simulink model "MMC_21_Level_Rectifier"  (R2023b)
settings: Solver=FixedStepAuto  StartTime=0.0  StopTime=0.5  RelTol=1e-3
libraries: spsSeriesRLCBranchLib x71, spsVoltageMeasurementLib x69, spsUniversalBridgeLib x60, spsCurrentMeasurementLib x8, slpidlib x7, spsRMSLib x3, spsACVoltageSourceLib x3, spsMeanLib x2, simulink x1, spsTHDLib x1, spspowerguiLib x1
(part 2 of 4)

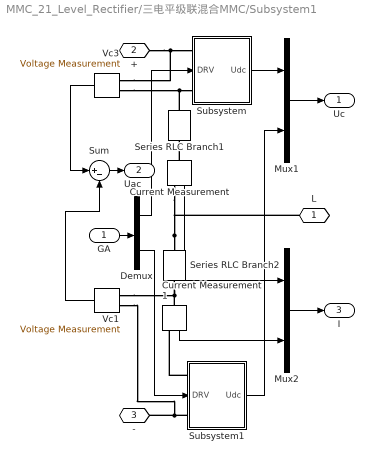
== system MMC_21_Level_Rectifier/三电平级联混合MMC/Subsystem1 ==
  GA : Inport
  Current Measurement : spsCurrentMeasurementLib/Current Measurement  PhasorSimulation=off  OutputType=Complex  PSBequivalent=0
  Current Measurement1 : spsCurrentMeasurementLib/Current Measurement  PhasorSimulation=off  OutputType=Complex  PSBequivalent=0
  Demux : Demux  Outputs=2
  Mux1 : Mux  Inputs=2
  Mux2 : Mux  Inputs=2
  Series RLC Branch1 : spsSeriesRLCBranchLib/Series RLC Branch  LConnTagsString=__new0  RConnTagsString=__new0  BranchType=L  Resistance=30  Inductance=1e-2  SetiL0=off  InitialCurrent=0  Capacitance=1e-6  Setx0=off  InitialVoltage=0  Measurements=None
  Series RLC Branch2 : spsSeriesRLCBranchLib/Series RLC Branch  LConnTagsString=__new0  RConnTagsString=__new0  BranchType=L  Resistance=30  Inductance=1e-2  SetiL0=off  InitialCurrent=0  Capacitance=1e-6  Setx0=off  InitialVoltage=0  Measurements=None
  Subsystem : Subsystem
      settings: PortSchema="{\"entries\":[{\"content\":{\"sides\":[{\"content\":{\"connectorIds\":[\"LConn1\",\"In1\",\"LConn2\"]},\"type\":\"ConnectorPlacement.EquallySpacedRectSide\",\"uuid\":\"6ff65170-2c54-424c-bb24-a96dc10d43f1\"},{\"content\":{\"connectorIds\":[\"Out1\"],\"side\":\"RIGHT\"},\"type\":\"ConnectorPlacement.EquallySpacedRectSide\",\"uuid\":\"90bd0adf-4df3-4011-8d6e-6638ef6b0231\"},{\"content\":{\"side\":\"TOP\"},\"type\":\"ConnectorPlacement.EquallySpacedRectSide\",\"uuid\":\"3c2ececc-9eb8-4d9a-8cd6-b7f9ee8fbc54\"}]},\"type\":\"ConnectorPlacement.EquallySpacedConnector\",\"uuid\":\"28e6b26b-947d-4977-abd9-a0ec0787b735\"}],\"packageUris\":[\"http://schema.mathworks.com/mf0/Connector/R2020b\"],\"version\":\"1.0\"}"
  Subsystem1 : Subsystem
      settings: PortSchema="{\"entries\":[{\"content\":{\"sides\":[{\"content\":{\"connectorIds\":[\"LConn1\",\"In1\",\"LConn2\"]},\"type\":\"ConnectorPlacement.EquallySpacedRectSide\",\"uuid\":\"6ff65170-2c54-424c-bb24-a96dc10d43f1\"},{\"content\":{\"connectorIds\":[\"Out1\"],\"side\":\"RIGHT\"},\"type\":\"ConnectorPlacement.EquallySpacedRectSide\",\"uuid\":\"90bd0adf-4df3-4011-8d6e-6638ef6b0231\"},{\"content\":{\"side\":\"TOP\"},\"type\":\"ConnectorPlacement.EquallySpacedRectSide\",\"uuid\":\"3c2ececc-9eb8-4d9a-8cd6-b7f9ee8fbc54\"}]},\"type\":\"ConnectorPlacement.EquallySpacedConnector\",\"uuid\":\"28e6b26b-947d-4977-abd9-a0ec0787b735\"}],\"packageUris\":[\"http://schema.mathworks.com/mf0/Connector/R2020b\"],\"version\":\"1.0\"}"
  Sum : Sum  Inputs=|+-
  Vc1 : spsVoltageMeasurementLib/Voltage Measurement  PhasorSimulation=off  OutputType=Complex  PSBequivalent=0
  Vc3 : spsVoltageMeasurementLib/Voltage Measurement  PhasorSimulation=off  OutputType=Complex  PSBequivalent=0
  L : PMIOPort  Side=Left
  + : PMIOPort  Port=2  Side=Left
  - : PMIOPort  Port=3  Side=Right
  Uc : Outport
  Uac : Outport  Port=2
  I : Outport  Port=3
  wires:
  Sum/1 -> Uac/1
  Vc1/1 -> Sum/2
  Vc3/1 -> Sum/1
  Mux2/1 -> I/1
  Current Measurement1/1 -> Mux2/2
  GA/1 -> Demux/1
  Demux/1 -> Subsystem/1(DRV)
  Current Measurement/1 -> Mux2/1
  Subsystem/1(Udc) -> Mux1/1
  Mux1/1 -> Uc/1
  Subsystem1/1(Udc) -> Mux1/2
  Demux/2 -> Subsystem1/1(DRV)
  connections:
  Vc1/LConn1 -- Series RLC Branch2/RConn1 -- Current Measurement1/LConn1
  Vc3/LConn1 -- +/RConn1 -- Subsystem/LConn1
  Vc1/LConn2 -- Subsystem1/LConn2 -- -/RConn1
  Current Measurement/LConn1 -- Series RLC Branch1/RConn1
  Subsystem1/LConn1 -- Current Measurement1/RConn1
  Subsystem/LConn2 -- Vc3/LConn2 -- Series RLC Branch1/LConn1
  Series RLC Branch2/LConn1 -- L/RConn1 -- Current Measurement/RConn1

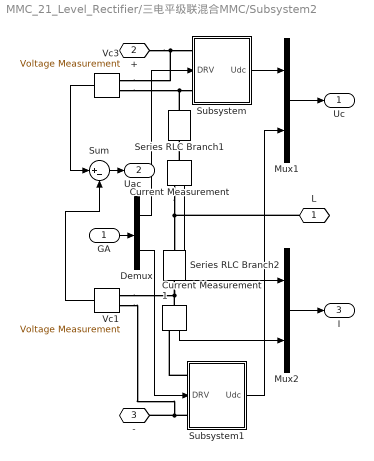
== system MMC_21_Level_Rectifier/三电平级联混合MMC/Subsystem2 ==
  GA : Inport
  Current Measurement : spsCurrentMeasurementLib/Current Measurement  PhasorSimulation=off  OutputType=Complex  PSBequivalent=0
  Current Measurement1 : spsCurrentMeasurementLib/Current Measurement  PhasorSimulation=off  OutputType=Complex  PSBequivalent=0
  Demux : Demux  Outputs=2
  Mux1 : Mux  Inputs=2
  Mux2 : Mux  Inputs=2
  Series RLC Branch1 : spsSeriesRLCBranchLib/Series RLC Branch  LConnTagsString=__new0  RConnTagsString=__new0  BranchType=L  Resistance=30  Inductance=1e-2  SetiL0=off  InitialCurrent=0  Capacitance=1e-6  Setx0=off  InitialVoltage=0  Measurements=None
  Series RLC Branch2 : spsSeriesRLCBranchLib/Series RLC Branch  LConnTagsString=__new0  RConnTagsString=__new0  BranchType=L  Resistance=30  Inductance=1e-2  SetiL0=off  InitialCurrent=0  Capacitance=1e-6  Setx0=off  InitialVoltage=0  Measurements=None
  Subsystem : Subsystem
      settings: PortSchema="{\"entries\":[{\"content\":{\"sides\":[{\"content\":{\"connectorIds\":[\"LConn1\",\"In1\",\"LConn2\"]},\"type\":\"ConnectorPlacement.EquallySpacedRectSide\",\"uuid\":\"6ff65170-2c54-424c-bb24-a96dc10d43f1\"},{\"content\":{\"connectorIds\":[\"Out1\"],\"side\":\"RIGHT\"},\"type\":\"ConnectorPlacement.EquallySpacedRectSide\",\"uuid\":\"90bd0adf-4df3-4011-8d6e-6638ef6b0231\"},{\"content\":{\"side\":\"TOP\"},\"type\":\"ConnectorPlacement.EquallySpacedRectSide\",\"uuid\":\"3c2ececc-9eb8-4d9a-8cd6-b7f9ee8fbc54\"}]},\"type\":\"ConnectorPlacement.EquallySpacedConnector\",\"uuid\":\"28e6b26b-947d-4977-abd9-a0ec0787b735\"}],\"packageUris\":[\"http://schema.mathworks.com/mf0/Connector/R2020b\"],\"version\":\"1.0\"}"
  Subsystem1 : Subsystem
      settings: PortSchema="{\"entries\":[{\"content\":{\"sides\":[{\"content\":{\"connectorIds\":[\"LConn1\",\"In1\",\"LConn2\"]},\"type\":\"ConnectorPlacement.EquallySpacedRectSide\",\"uuid\":\"6ff65170-2c54-424c-bb24-a96dc10d43f1\"},{\"content\":{\"connectorIds\":[\"Out1\"],\"side\":\"RIGHT\"},\"type\":\"ConnectorPlacement.EquallySpacedRectSide\",\"uuid\":\"90bd0adf-4df3-4011-8d6e-6638ef6b0231\"},{\"content\":{\"side\":\"TOP\"},\"type\":\"ConnectorPlacement.EquallySpacedRectSide\",\"uuid\":\"3c2ececc-9eb8-4d9a-8cd6-b7f9ee8fbc54\"}]},\"type\":\"ConnectorPlacement.EquallySpacedConnector\",\"uuid\":\"28e6b26b-947d-4977-abd9-a0ec0787b735\"}],\"packageUris\":[\"http://schema.mathworks.com/mf0/Connector/R2020b\"],\"version\":\"1.0\"}"
  Sum : Sum  Inputs=|+-
  Vc1 : spsVoltageMeasurementLib/Voltage Measurement  PhasorSimulation=off  OutputType=Complex  PSBequivalent=0
  Vc3 : spsVoltageMeasurementLib/Voltage Measurement  PhasorSimulation=off  OutputType=Complex  PSBequivalent=0
  L : PMIOPort  Side=Left
  + : PMIOPort  Port=2  Side=Left
  - : PMIOPort  Port=3  Side=Right
  Uc : Outport
  Uac : Outport  Port=2
  I : Outport  Port=3
  wires:
  Demux/2 -> Subsystem1/1(DRV)
  Subsystem1/1(Udc) -> Mux1/2
  Mux1/1 -> Uc/1
  Subsystem/1(Udc) -> Mux1/1
  Current Measurement/1 -> Mux2/1
  Demux/1 -> Subsystem/1(DRV)
  GA/1 -> Demux/1
  Current Measurement1/1 -> Mux2/2
  Mux2/1 -> I/1
  Vc3/1 -> Sum/1
  Vc1/1 -> Sum/2
  Sum/1 -> Uac/1
  connections:
  Current Measurement/RConn1 -- Series RLC Branch2/LConn1 -- L/RConn1
  Series RLC Branch1/LConn1 -- Vc3/LConn2 -- Subsystem/LConn2
  Subsystem1/LConn1 -- Current Measurement1/RConn1
  Current Measurement/LConn1 -- Series RLC Branch1/RConn1
  Subsystem1/LConn2 -- Vc1/LConn2 -- -/RConn1
  +/RConn1 -- Vc3/LConn1 -- Subsystem/LConn1
  Current Measurement1/LConn1 -- Vc1/LConn1 -- Series RLC Branch2/RConn1

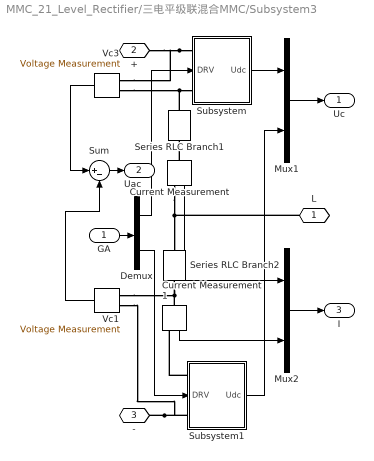
== system MMC_21_Level_Rectifier/三电平级联混合MMC/Subsystem3 ==
  GA : Inport
  Current Measurement : spsCurrentMeasurementLib/Current Measurement  PhasorSimulation=off  OutputType=Complex  PSBequivalent=0
  Current Measurement1 : spsCurrentMeasurementLib/Current Measurement  PhasorSimulation=off  OutputType=Complex  PSBequivalent=0
  Demux : Demux  Outputs=2
  Mux1 : Mux  Inputs=2
  Mux2 : Mux  Inputs=2
  Series RLC Branch1 : spsSeriesRLCBranchLib/Series RLC Branch  LConnTagsString=__new0  RConnTagsString=__new0  BranchType=L  Resistance=30  Inductance=1e-2  SetiL0=off  InitialCurrent=0  Capacitance=1e-6  Setx0=off  InitialVoltage=0  Measurements=None
  Series RLC Branch2 : spsSeriesRLCBranchLib/Series RLC Branch  LConnTagsString=__new0  RConnTagsString=__new0  BranchType=L  Resistance=30  Inductance=1e-2  SetiL0=off  InitialCurrent=0  Capacitance=1e-6  Setx0=off  InitialVoltage=0  Measurements=None
  Subsystem : Subsystem
      settings: PortSchema="{\"entries\":[{\"content\":{\"sides\":[{\"content\":{\"connectorIds\":[\"LConn1\",\"In1\",\"LConn2\"]},\"type\":\"ConnectorPlacement.EquallySpacedRectSide\",\"uuid\":\"6ff65170-2c54-424c-bb24-a96dc10d43f1\"},{\"content\":{\"connectorIds\":[\"Out1\"],\"side\":\"RIGHT\"},\"type\":\"ConnectorPlacement.EquallySpacedRectSide\",\"uuid\":\"90bd0adf-4df3-4011-8d6e-6638ef6b0231\"},{\"content\":{\"side\":\"TOP\"},\"type\":\"ConnectorPlacement.EquallySpacedRectSide\",\"uuid\":\"3c2ececc-9eb8-4d9a-8cd6-b7f9ee8fbc54\"}]},\"type\":\"ConnectorPlacement.EquallySpacedConnector\",\"uuid\":\"28e6b26b-947d-4977-abd9-a0ec0787b735\"}],\"packageUris\":[\"http://schema.mathworks.com/mf0/Connector/R2020b\"],\"version\":\"1.0\"}"
  Subsystem1 : Subsystem
      settings: PortSchema="{\"entries\":[{\"content\":{\"sides\":[{\"content\":{\"connectorIds\":[\"LConn1\",\"In1\",\"LConn2\"]},\"type\":\"ConnectorPlacement.EquallySpacedRectSide\",\"uuid\":\"6ff65170-2c54-424c-bb24-a96dc10d43f1\"},{\"content\":{\"connectorIds\":[\"Out1\"],\"side\":\"RIGHT\"},\"type\":\"ConnectorPlacement.EquallySpacedRectSide\",\"uuid\":\"90bd0adf-4df3-4011-8d6e-6638ef6b0231\"},{\"content\":{\"side\":\"TOP\"},\"type\":\"ConnectorPlacement.EquallySpacedRectSide\",\"uuid\":\"3c2ececc-9eb8-4d9a-8cd6-b7f9ee8fbc54\"}]},\"type\":\"ConnectorPlacement.EquallySpacedConnector\",\"uuid\":\"28e6b26b-947d-4977-abd9-a0ec0787b735\"}],\"packageUris\":[\"http://schema.mathworks.com/mf0/Connector/R2020b\"],\"version\":\"1.0\"}"
  Sum : Sum  Inputs=|+-
  Vc1 : spsVoltageMeasurementLib/Voltage Measurement  PhasorSimulation=off  OutputType=Complex  PSBequivalent=0
  Vc3 : spsVoltageMeasurementLib/Voltage Measurement  PhasorSimulation=off  OutputType=Complex  PSBequivalent=0
  L : PMIOPort  Side=Left
  + : PMIOPort  Port=2  Side=Left
  - : PMIOPort  Port=3  Side=Right
  Uc : Outport
  Uac : Outport  Port=2
  I : Outport  Port=3
  wires:
  Demux/2 -> Subsystem1/1(DRV)
  Subsystem1/1(Udc) -> Mux1/2
  Mux1/1 -> Uc/1
  Subsystem/1(Udc) -> Mux1/1
  Current Measurement/1 -> Mux2/1
  Demux/1 -> Subsystem/1(DRV)
  GA/1 -> Demux/1
  Current Measurement1/1 -> Mux2/2
  Mux2/1 -> I/1
  Vc3/1 -> Sum/1
  Vc1/1 -> Sum/2
  Sum/1 -> Uac/1
  connections:
  Current Measurement/RConn1 -- L/RConn1 -- Series RLC Branch2/LConn1
  Series RLC Branch1/LConn1 -- Vc3/LConn2 -- Subsystem/LConn2
  Subsystem1/LConn1 -- Current Measurement1/RConn1
  Current Measurement/LConn1 -- Series RLC Branch1/RConn1
  -/RConn1 -- Subsystem1/LConn2 -- Vc1/LConn2
  Subsystem/LConn1 -- +/RConn1 -- Vc3/LConn1
  Current Measurement1/LConn1 -- Series RLC Branch2/RConn1 -- Vc1/LConn1

== system MMC_21_Level_Rectifier/准PR电压电流环路/2//3 Transform ==
  ac : Inport
  Demux : Demux  Outputs=2
  Mux : Mux  Inputs=3
  Sum1 : Sum  Inputs=-|-
  abc : Outport
  wires:
  Sum1/1 -> Mux/2
  Mux/1 -> abc/1
  Demux/1 -> Sum1/1, Mux/1
  ac/1 -> Demux/1
  Demux/2 -> Sum1/2, Mux/3

== system MMC_21_Level_Rectifier/准PR电压电流环路/Digital PR A-C ==
  err : Inport
  Constant : Constant  Value=Kp
  Constant1 : Constant  Value=Kr
  Constant2 : Constant  Value=Wc
  Constant3 : Constant  Value=Ts
  Demux : Demux  Outputs=2
  Discrete PR : MATLAB Function  TreatAsAtomicUnit=on
  Mux : Mux  Inputs=2
  Saturation : Saturate  UpperLimit=Upper  LowerLimit=Lower
  out : Outport
  wires:
  Constant1/1 -> Discrete PR/4(Kr)
  Constant3/1 -> Discrete PR/6(Ts)
  Constant/1 -> Discrete PR/3(Kp)
  Constant2/1 -> Discrete PR/5(Wc)
  Demux/1 -> Discrete PR/1(err_A)
  err/1 -> Demux/1
  Demux/2 -> Discrete PR/2(err_C)
  Discrete PR/1(out_A) -> Mux/1
  Discrete PR/2(out_C) -> Mux/2
  Mux/1 -> Saturation/1
  Saturation/1 -> out/1

== system MMC_21_Level_Rectifier/三电平级联混合MMC/Subsystem1/Subsystem ==
  DRV : Inport
  Demux1 : Demux  Outputs=5
  Mux1 : Mux  Inputs=5
  混合三电平子模块1 : Subsystem
      settings: PortSchema="{\"entries\":[{\"content\":{\"sides\":[{\"content\":{\"connectorIds\":[\"LConn1\",\"In1\",\"LConn2\"]},\"type\":\"ConnectorPlacement.EquallySpacedRectSide\",\"uuid\":\"9e595762-cb5d-4bdb-b148-c61b2a1e03b2\"},{\"content\":{\"connectorIds\":[\"Out1\"],\"side\":\"RIGHT\"},\"type\":\"ConnectorPlacement.EquallySpacedRectSide\",\"uuid\":\"493db82a-06a2-4a87-b234-4e7c0dd8f89b\"},{\"content\":{\"side\":\"TOP\"},\"type\":\"ConnectorPlacement.EquallySpacedRectSide\",\"uuid\":\"00eff750-16ab-4a5d-887e-7c480e5e0d14\"}]},\"type\":\"ConnectorPlacement.EquallySpacedConnector\",\"uuid\":\"9358f970-c1dc-48f9-b6f8-bcc3c6345ab1\"}],\"packageUris\":[\"http://schema.mathworks.com/mf0/Connector/R2020b\"],\"version\":\"1.0\"}"
  混合三电平子模块2 : Subsystem
      settings: PortSchema="{\"entries\":[{\"content\":{\"sides\":[{\"content\":{\"connectorIds\":[\"LConn1\",\"In1\",\"LConn2\"]},\"type\":\"ConnectorPlacement.EquallySpacedRectSide\",\"uuid\":\"9e595762-cb5d-4bdb-b148-c61b2a1e03b2\"},{\"content\":{\"connectorIds\":[\"Out1\"],\"side\":\"RIGHT\"},\"type\":\"ConnectorPlacement.EquallySpacedRectSide\",\"uuid\":\"493db82a-06a2-4a87-b234-4e7c0dd8f89b\"},{\"content\":{\"side\":\"TOP\"},\"type\":\"ConnectorPlacement.EquallySpacedRectSide\",\"uuid\":\"00eff750-16ab-4a5d-887e-7c480e5e0d14\"}]},\"type\":\"ConnectorPlacement.EquallySpacedConnector\",\"uuid\":\"9358f970-c1dc-48f9-b6f8-bcc3c6345ab1\"}],\"packageUris\":[\"http://schema.mathworks.com/mf0/Connector/R2020b\"],\"version\":\"1.0\"}"
  混合三电平子模块3 : Subsystem
      settings: PortSchema="{\"entries\":[{\"content\":{\"sides\":[{\"content\":{\"connectorIds\":[\"LConn1\",\"In1\",\"LConn2\"]},\"type\":\"ConnectorPlacement.EquallySpacedRectSide\",\"uuid\":\"9e595762-cb5d-4bdb-b148-c61b2a1e03b2\"},{\"content\":{\"connectorIds\":[\"Out1\"],\"side\":\"RIGHT\"},\"type\":\"ConnectorPlacement.EquallySpacedRectSide\",\"uuid\":\"493db82a-06a2-4a87-b234-4e7c0dd8f89b\"},{\"content\":{\"side\":\"TOP\"},\"type\":\"ConnectorPlacement.EquallySpacedRectSide\",\"uuid\":\"00eff750-16ab-4a5d-887e-7c480e5e0d14\"}]},\"type\":\"ConnectorPlacement.EquallySpacedConnector\",\"uuid\":\"9358f970-c1dc-48f9-b6f8-bcc3c6345ab1\"}],\"packageUris\":[\"http://schema.mathworks.com/mf0/Connector/R2020b\"],\"version\":\"1.0\"}"
  混合三电平子模块4 : Subsystem
      settings: PortSchema="{\"entries\":[{\"content\":{\"sides\":[{\"content\":{\"connectorIds\":[\"LConn1\",\"In1\",\"LConn2\"]},\"type\":\"ConnectorPlacement.EquallySpacedRectSide\",\"uuid\":\"9e595762-cb5d-4bdb-b148-c61b2a1e03b2\"},{\"content\":{\"connectorIds\":[\"Out1\"],\"side\":\"RIGHT\"},\"type\":\"ConnectorPlacement.EquallySpacedRectSide\",\"uuid\":\"493db82a-06a2-4a87-b234-4e7c0dd8f89b\"},{\"content\":{\"side\":\"TOP\"},\"type\":\"ConnectorPlacement.EquallySpacedRectSide\",\"uuid\":\"00eff750-16ab-4a5d-887e-7c480e5e0d14\"}]},\"type\":\"ConnectorPlacement.EquallySpacedConnector\",\"uuid\":\"9358f970-c1dc-48f9-b6f8-bcc3c6345ab1\"}],\"packageUris\":[\"http://schema.mathworks.com/mf0/Connector/R2020b\"],\"version\":\"1.0\"}"
  混合三电平子模块5 : Subsystem
      settings: PortSchema="{\"entries\":[{\"content\":{\"sides\":[{\"content\":{\"connectorIds\":[\"LConn1\",\"In1\",\"LConn2\"]},\"type\":\"ConnectorPlacement.EquallySpacedRectSide\",\"uuid\":\"9e595762-cb5d-4bdb-b148-c61b2a1e03b2\"},{\"content\":{\"connectorIds\":[\"Out1\"],\"side\":\"RIGHT\"},\"type\":\"ConnectorPlacement.EquallySpacedRectSide\",\"uuid\":\"493db82a-06a2-4a87-b234-4e7c0dd8f89b\"},{\"content\":{\"side\":\"TOP\"},\"type\":\"ConnectorPlacement.EquallySpacedRectSide\",\"uuid\":\"00eff750-16ab-4a5d-887e-7c480e5e0d14\"}]},\"type\":\"ConnectorPlacement.EquallySpacedConnector\",\"uuid\":\"9358f970-c1dc-48f9-b6f8-bcc3c6345ab1\"}],\"packageUris\":[\"http://schema.mathworks.com/mf0/Connector/R2020b\"],\"version\":\"1.0\"}"
  + : PMIOPort  Side=Left
  - : PMIOPort  Port=2  Side=Left
  Udc : Outport
  wires:
  混合三电平子模块1/1(Udc) -> Mux1/1
  Mux1/1 -> Udc/1
  混合三电平子模块5/1(Udc) -> Mux1/5
  混合三电平子模块4/1(Udc) -> Mux1/4
  混合三电平子模块2/1(Udc) -> Mux1/2
  混合三电平子模块3/1(Udc) -> Mux1/3
  Demux1/5 -> 混合三电平子模块5/1(DRV)
  Demux1/4 -> 混合三电平子模块4/1(DRV)
  Demux1/2 -> 混合三电平子模块2/1(DRV)
  Demux1/3 -> 混合三电平子模块3/1(DRV)
  Demux1/1 -> 混合三电平子模块1/1(DRV)
  DRV/1 -> Demux1/1
  connections:
  混合三电平子模块5/LConn1 -- 混合三电平子模块4/LConn2
  混合三电平子模块4/LConn1 -- 混合三电平子模块3/LConn2
  混合三电平子模块3/LConn1 -- 混合三电平子模块2/LConn2
  混合三电平子模块2/LConn1 -- 混合三电平子模块1/LConn2
  +/RConn1 -- 混合三电平子模块1/LConn1
  混合三电平子模块5/LConn2 -- -/RConn1

== system MMC_21_Level_Rectifier/三电平级联混合MMC/Subsystem1/Subsystem1 ==
  DRV : Inport
  Demux1 : Demux  Outputs=5
  Mux1 : Mux  Inputs=5
  混合三电平子模块1 : Subsystem
      settings: PortSchema="{\"entries\":[{\"content\":{\"sides\":[{\"content\":{\"connectorIds\":[\"LConn1\",\"In1\",\"LConn2\"]},\"type\":\"ConnectorPlacement.EquallySpacedRectSide\",\"uuid\":\"9e595762-cb5d-4bdb-b148-c61b2a1e03b2\"},{\"content\":{\"connectorIds\":[\"Out1\"],\"side\":\"RIGHT\"},\"type\":\"ConnectorPlacement.EquallySpacedRectSide\",\"uuid\":\"493db82a-06a2-4a87-b234-4e7c0dd8f89b\"},{\"content\":{\"side\":\"TOP\"},\"type\":\"ConnectorPlacement.EquallySpacedRectSide\",\"uuid\":\"00eff750-16ab-4a5d-887e-7c480e5e0d14\"}]},\"type\":\"ConnectorPlacement.EquallySpacedConnector\",\"uuid\":\"9358f970-c1dc-48f9-b6f8-bcc3c6345ab1\"}],\"packageUris\":[\"http://schema.mathworks.com/mf0/Connector/R2020b\"],\"version\":\"1.0\"}"
  混合三电平子模块2 : Subsystem
      settings: PortSchema="{\"entries\":[{\"content\":{\"sides\":[{\"content\":{\"connectorIds\":[\"LConn1\",\"In1\",\"LConn2\"]},\"type\":\"ConnectorPlacement.EquallySpacedRectSide\",\"uuid\":\"9e595762-cb5d-4bdb-b148-c61b2a1e03b2\"},{\"content\":{\"connectorIds\":[\"Out1\"],\"side\":\"RIGHT\"},\"type\":\"ConnectorPlacement.EquallySpacedRectSide\",\"uuid\":\"493db82a-06a2-4a87-b234-4e7c0dd8f89b\"},{\"content\":{\"side\":\"TOP\"},\"type\":\"ConnectorPlacement.EquallySpacedRectSide\",\"uuid\":\"00eff750-16ab-4a5d-887e-7c480e5e0d14\"}]},\"type\":\"ConnectorPlacement.EquallySpacedConnector\",\"uuid\":\"9358f970-c1dc-48f9-b6f8-bcc3c6345ab1\"}],\"packageUris\":[\"http://schema.mathworks.com/mf0/Connector/R2020b\"],\"version\":\"1.0\"}"
  混合三电平子模块3 : Subsystem
      settings: PortSchema="{\"entries\":[{\"content\":{\"sides\":[{\"content\":{\"connectorIds\":[\"LConn1\",\"In1\",\"LConn2\"]},\"type\":\"ConnectorPlacement.EquallySpacedRectSide\",\"uuid\":\"9e595762-cb5d-4bdb-b148-c61b2a1e03b2\"},{\"content\":{\"connectorIds\":[\"Out1\"],\"side\":\"RIGHT\"},\"type\":\"ConnectorPlacement.EquallySpacedRectSide\",\"uuid\":\"493db82a-06a2-4a87-b234-4e7c0dd8f89b\"},{\"content\":{\"side\":\"TOP\"},\"type\":\"ConnectorPlacement.EquallySpacedRectSide\",\"uuid\":\"00eff750-16ab-4a5d-887e-7c480e5e0d14\"}]},\"type\":\"ConnectorPlacement.EquallySpacedConnector\",\"uuid\":\"9358f970-c1dc-48f9-b6f8-bcc3c6345ab1\"}],\"packageUris\":[\"http://schema.mathworks.com/mf0/Connector/R2020b\"],\"version\":\"1.0\"}"
  混合三电平子模块4 : Subsystem
      settings: PortSchema="{\"entries\":[{\"content\":{\"sides\":[{\"content\":{\"connectorIds\":[\"LConn1\",\"In1\",\"LConn2\"]},\"type\":\"ConnectorPlacement.EquallySpacedRectSide\",\"uuid\":\"9e595762-cb5d-4bdb-b148-c61b2a1e03b2\"},{\"content\":{\"connectorIds\":[\"Out1\"],\"side\":\"RIGHT\"},\"type\":\"ConnectorPlacement.EquallySpacedRectSide\",\"uuid\":\"493db82a-06a2-4a87-b234-4e7c0dd8f89b\"},{\"content\":{\"side\":\"TOP\"},\"type\":\"ConnectorPlacement.EquallySpacedRectSide\",\"uuid\":\"00eff750-16ab-4a5d-887e-7c480e5e0d14\"}]},\"type\":\"ConnectorPlacement.EquallySpacedConnector\",\"uuid\":\"9358f970-c1dc-48f9-b6f8-bcc3c6345ab1\"}],\"packageUris\":[\"http://schema.mathworks.com/mf0/Connector/R2020b\"],\"version\":\"1.0\"}"
  混合三电平子模块5 : Subsystem
      settings: PortSchema="{\"entries\":[{\"content\":{\"sides\":[{\"content\":{\"connectorIds\":[\"LConn1\",\"In1\",\"LConn2\"]},\"type\":\"ConnectorPlacement.EquallySpacedRectSide\",\"uuid\":\"9e595762-cb5d-4bdb-b148-c61b2a1e03b2\"},{\"content\":{\"connectorIds\":[\"Out1\"],\"side\":\"RIGHT\"},\"type\":\"ConnectorPlacement.EquallySpacedRectSide\",\"uuid\":\"493db82a-06a2-4a87-b234-4e7c0dd8f89b\"},{\"content\":{\"side\":\"TOP\"},\"type\":\"ConnectorPlacement.EquallySpacedRectSide\",\"uuid\":\"00eff750-16ab-4a5d-887e-7c480e5e0d14\"}]},\"type\":\"ConnectorPlacement.EquallySpacedConnector\",\"uuid\":\"9358f970-c1dc-48f9-b6f8-bcc3c6345ab1\"}],\"packageUris\":[\"http://schema.mathworks.com/mf0/Connector/R2020b\"],\"version\":\"1.0\"}"
  + : PMIOPort  Side=Left
  - : PMIOPort  Port=2  Side=Left
  Udc : Outport
  wires:
  DRV/1 -> Demux1/1
  Demux1/1 -> 混合三电平子模块1/1(DRV)
  Demux1/3 -> 混合三电平子模块3/1(DRV)
  Demux1/2 -> 混合三电平子模块2/1(DRV)
  Demux1/4 -> 混合三电平子模块4/1(DRV)
  Demux1/5 -> 混合三电平子模块5/1(DRV)
  混合三电平子模块3/1(Udc) -> Mux1/3
  混合三电平子模块2/1(Udc) -> Mux1/2
  混合三电平子模块4/1(Udc) -> Mux1/4
  混合三电平子模块5/1(Udc) -> Mux1/5
  Mux1/1 -> Udc/1
  混合三电平子模块1/1(Udc) -> Mux1/1
  connections:
  混合三电平子模块5/LConn2 -- -/RConn1
  +/RConn1 -- 混合三电平子模块1/LConn1
  混合三电平子模块2/LConn1 -- 混合三电平子模块1/LConn2
  混合三电平子模块3/LConn1 -- 混合三电平子模块2/LConn2
  混合三电平子模块4/LConn1 -- 混合三电平子模块3/LConn2
  混合三电平子模块5/LConn1 -- 混合三电平子模块4/LConn2

== system MMC_21_Level_Rectifier/三电平级联混合MMC/Subsystem2/Subsystem ==
  DRV : Inport
  Demux1 : Demux  Outputs=5
  Mux1 : Mux  Inputs=5
  混合三电平子模块1 : Subsystem
      settings: PortSchema="{\"entries\":[{\"content\":{\"sides\":[{\"content\":{\"connectorIds\":[\"LConn1\",\"In1\",\"LConn2\"]},\"type\":\"ConnectorPlacement.EquallySpacedRectSide\",\"uuid\":\"9e595762-cb5d-4bdb-b148-c61b2a1e03b2\"},{\"content\":{\"connectorIds\":[\"Out1\"],\"side\":\"RIGHT\"},\"type\":\"ConnectorPlacement.EquallySpacedRectSide\",\"uuid\":\"493db82a-06a2-4a87-b234-4e7c0dd8f89b\"},{\"content\":{\"side\":\"TOP\"},\"type\":\"ConnectorPlacement.EquallySpacedRectSide\",\"uuid\":\"00eff750-16ab-4a5d-887e-7c480e5e0d14\"}]},\"type\":\"ConnectorPlacement.EquallySpacedConnector\",\"uuid\":\"9358f970-c1dc-48f9-b6f8-bcc3c6345ab1\"}],\"packageUris\":[\"http://schema.mathworks.com/mf0/Connector/R2020b\"],\"version\":\"1.0\"}"
  混合三电平子模块2 : Subsystem
      settings: PortSchema="{\"entries\":[{\"content\":{\"sides\":[{\"content\":{\"connectorIds\":[\"LConn1\",\"In1\",\"LConn2\"]},\"type\":\"ConnectorPlacement.EquallySpacedRectSide\",\"uuid\":\"9e595762-cb5d-4bdb-b148-c61b2a1e03b2\"},{\"content\":{\"connectorIds\":[\"Out1\"],\"side\":\"RIGHT\"},\"type\":\"ConnectorPlacement.EquallySpacedRectSide\",\"uuid\":\"493db82a-06a2-4a87-b234-4e7c0dd8f89b\"},{\"content\":{\"side\":\"TOP\"},\"type\":\"ConnectorPlacement.EquallySpacedRectSide\",\"uuid\":\"00eff750-16ab-4a5d-887e-7c480e5e0d14\"}]},\"type\":\"ConnectorPlacement.EquallySpacedConnector\",\"uuid\":\"9358f970-c1dc-48f9-b6f8-bcc3c6345ab1\"}],\"packageUris\":[\"http://schema.mathworks.com/mf0/Connector/R2020b\"],\"version\":\"1.0\"}"
  混合三电平子模块3 : Subsystem
      settings: PortSchema="{\"entries\":[{\"content\":{\"sides\":[{\"content\":{\"connectorIds\":[\"LConn1\",\"In1\",\"LConn2\"]},\"type\":\"ConnectorPlacement.EquallySpacedRectSide\",\"uuid\":\"9e595762-cb5d-4bdb-b148-c61b2a1e03b2\"},{\"content\":{\"connectorIds\":[\"Out1\"],\"side\":\"RIGHT\"},\"type\":\"ConnectorPlacement.EquallySpacedRectSide\",\"uuid\":\"493db82a-06a2-4a87-b234-4e7c0dd8f89b\"},{\"content\":{\"side\":\"TOP\"},\"type\":\"ConnectorPlacement.EquallySpacedRectSide\",\"uuid\":\"00eff750-16ab-4a5d-887e-7c480e5e0d14\"}]},\"type\":\"ConnectorPlacement.EquallySpacedConnector\",\"uuid\":\"9358f970-c1dc-48f9-b6f8-bcc3c6345ab1\"}],\"packageUris\":[\"http://schema.mathworks.com/mf0/Connector/R2020b\"],\"version\":\"1.0\"}"
  混合三电平子模块4 : Subsystem
      settings: PortSchema="{\"entries\":[{\"content\":{\"sides\":[{\"content\":{\"connectorIds\":[\"LConn1\",\"In1\",\"LConn2\"]},\"type\":\"ConnectorPlacement.EquallySpacedRectSide\",\"uuid\":\"9e595762-cb5d-4bdb-b148-c61b2a1e03b2\"},{\"content\":{\"connectorIds\":[\"Out1\"],\"side\":\"RIGHT\"},\"type\":\"ConnectorPlacement.EquallySpacedRectSide\",\"uuid\":\"493db82a-06a2-4a87-b234-4e7c0dd8f89b\"},{\"content\":{\"side\":\"TOP\"},\"type\":\"ConnectorPlacement.EquallySpacedRectSide\",\"uuid\":\"00eff750-16ab-4a5d-887e-7c480e5e0d14\"}]},\"type\":\"ConnectorPlacement.EquallySpacedConnector\",\"uuid\":\"9358f970-c1dc-48f9-b6f8-bcc3c6345ab1\"}],\"packageUris\":[\"http://schema.mathworks.com/mf0/Connector/R2020b\"],\"version\":\"1.0\"}"
  混合三电平子模块5 : Subsystem
      settings: PortSchema="{\"entries\":[{\"content\":{\"sides\":[{\"content\":{\"connectorIds\":[\"LConn1\",\"In1\",\"LConn2\"]},\"type\":\"ConnectorPlacement.EquallySpacedRectSide\",\"uuid\":\"9e595762-cb5d-4bdb-b148-c61b2a1e03b2\"},{\"content\":{\"connectorIds\":[\"Out1\"],\"side\":\"RIGHT\"},\"type\":\"ConnectorPlacement.EquallySpacedRectSide\",\"uuid\":\"493db82a-06a2-4a87-b234-4e7c0dd8f89b\"},{\"content\":{\"side\":\"TOP\"},\"type\":\"ConnectorPlacement.EquallySpacedRectSide\",\"uuid\":\"00eff750-16ab-4a5d-887e-7c480e5e0d14\"}]},\"type\":\"ConnectorPlacement.EquallySpacedConnector\",\"uuid\":\"9358f970-c1dc-48f9-b6f8-bcc3c6345ab1\"}],\"packageUris\":[\"http://schema.mathworks.com/mf0/Connector/R2020b\"],\"version\":\"1.0\"}"
  + : PMIOPort  Side=Left
  - : PMIOPort  Port=2  Side=Left
  Udc : Outport
  wires:
  DRV/1 -> Demux1/1
  Demux1/1 -> 混合三电平子模块1/1(DRV)
  Demux1/3 -> 混合三电平子模块3/1(DRV)
  Demux1/2 -> 混合三电平子模块2/1(DRV)
  Demux1/4 -> 混合三电平子模块4/1(DRV)
  Demux1/5 -> 混合三电平子模块5/1(DRV)
  混合三电平子模块3/1(Udc) -> Mux1/3
  混合三电平子模块2/1(Udc) -> Mux1/2
  混合三电平子模块4/1(Udc) -> Mux1/4
  混合三电平子模块5/1(Udc) -> Mux1/5
  Mux1/1 -> Udc/1
  混合三电平子模块1/1(Udc) -> Mux1/1
  connections:
  混合三电平子模块5/LConn2 -- -/RConn1
  +/RConn1 -- 混合三电平子模块1/LConn1
  混合三电平子模块2/LConn1 -- 混合三电平子模块1/LConn2
  混合三电平子模块3/LConn1 -- 混合三电平子模块2/LConn2
  混合三电平子模块4/LConn1 -- 混合三电平子模块3/LConn2
  混合三电平子模块5/LConn1 -- 混合三电平子模块4/LConn2

== system MMC_21_Level_Rectifier/三电平级联混合MMC/Subsystem2/Subsystem1 ==
  DRV : Inport
  Demux1 : Demux  Outputs=5
  Mux1 : Mux  Inputs=5
  混合三电平子模块1 : Subsystem
      settings: PortSchema="{\"entries\":[{\"content\":{\"sides\":[{\"content\":{\"connectorIds\":[\"LConn1\",\"In1\",\"LConn2\"]},\"type\":\"ConnectorPlacement.EquallySpacedRectSide\",\"uuid\":\"9e595762-cb5d-4bdb-b148-c61b2a1e03b2\"},{\"content\":{\"connectorIds\":[\"Out1\"],\"side\":\"RIGHT\"},\"type\":\"ConnectorPlacement.EquallySpacedRectSide\",\"uuid\":\"493db82a-06a2-4a87-b234-4e7c0dd8f89b\"},{\"content\":{\"side\":\"TOP\"},\"type\":\"ConnectorPlacement.EquallySpacedRectSide\",\"uuid\":\"00eff750-16ab-4a5d-887e-7c480e5e0d14\"}]},\"type\":\"ConnectorPlacement.EquallySpacedConnector\",\"uuid\":\"9358f970-c1dc-48f9-b6f8-bcc3c6345ab1\"}],\"packageUris\":[\"http://schema.mathworks.com/mf0/Connector/R2020b\"],\"version\":\"1.0\"}"
  混合三电平子模块2 : Subsystem
      settings: PortSchema="{\"entries\":[{\"content\":{\"sides\":[{\"content\":{\"connectorIds\":[\"LConn1\",\"In1\",\"LConn2\"]},\"type\":\"ConnectorPlacement.EquallySpacedRectSide\",\"uuid\":\"9e595762-cb5d-4bdb-b148-c61b2a1e03b2\"},{\"content\":{\"connectorIds\":[\"Out1\"],\"side\":\"RIGHT\"},\"type\":\"ConnectorPlacement.EquallySpacedRectSide\",\"uuid\":\"493db82a-06a2-4a87-b234-4e7c0dd8f89b\"},{\"content\":{\"side\":\"TOP\"},\"type\":\"ConnectorPlacement.EquallySpacedRectSide\",\"uuid\":\"00eff750-16ab-4a5d-887e-7c480e5e0d14\"}]},\"type\":\"ConnectorPlacement.EquallySpacedConnector\",\"uuid\":\"9358f970-c1dc-48f9-b6f8-bcc3c6345ab1\"}],\"packageUris\":[\"http://schema.mathworks.com/mf0/Connector/R2020b\"],\"version\":\"1.0\"}"
  混合三电平子模块3 : Subsystem
      settings: PortSchema="{\"entries\":[{\"content\":{\"sides\":[{\"content\":{\"connectorIds\":[\"LConn1\",\"In1\",\"LConn2\"]},\"type\":\"ConnectorPlacement.EquallySpacedRectSide\",\"uuid\":\"9e595762-cb5d-4bdb-b148-c61b2a1e03b2\"},{\"content\":{\"connectorIds\":[\"Out1\"],\"side\":\"RIGHT\"},\"type\":\"ConnectorPlacement.EquallySpacedRectSide\",\"uuid\":\"493db82a-06a2-4a87-b234-4e7c0dd8f89b\"},{\"content\":{\"side\":\"TOP\"},\"type\":\"ConnectorPlacement.EquallySpacedRectSide\",\"uuid\":\"00eff750-16ab-4a5d-887e-7c480e5e0d14\"}]},\"type\":\"ConnectorPlacement.EquallySpacedConnector\",\"uuid\":\"9358f970-c1dc-48f9-b6f8-bcc3c6345ab1\"}],\"packageUris\":[\"http://schema.mathworks.com/mf0/Connector/R2020b\"],\"version\":\"1.0\"}"
  混合三电平子模块4 : Subsystem
      settings: PortSchema="{\"entries\":[{\"content\":{\"sides\":[{\"content\":{\"connectorIds\":[\"LConn1\",\"In1\",\"LConn2\"]},\"type\":\"ConnectorPlacement.EquallySpacedRectSide\",\"uuid\":\"9e595762-cb5d-4bdb-b148-c61b2a1e03b2\"},{\"content\":{\"connectorIds\":[\"Out1\"],\"side\":\"RIGHT\"},\"type\":\"ConnectorPlacement.EquallySpacedRectSide\",\"uuid\":\"493db82a-06a2-4a87-b234-4e7c0dd8f89b\"},{\"content\":{\"side\":\"TOP\"},\"type\":\"ConnectorPlacement.EquallySpacedRectSide\",\"uuid\":\"00eff750-16ab-4a5d-887e-7c480e5e0d14\"}]},\"type\":\"ConnectorPlacement.EquallySpacedConnector\",\"uuid\":\"9358f970-c1dc-48f9-b6f8-bcc3c6345ab1\"}],\"packageUris\":[\"http://schema.mathworks.com/mf0/Connector/R2020b\"],\"version\":\"1.0\"}"
  混合三电平子模块5 : Subsystem
      settings: PortSchema="{\"entries\":[{\"content\":{\"sides\":[{\"content\":{\"connectorIds\":[\"LConn1\",\"In1\",\"LConn2\"]},\"type\":\"ConnectorPlacement.EquallySpacedRectSide\",\"uuid\":\"9e595762-cb5d-4bdb-b148-c61b2a1e03b2\"},{\"content\":{\"connectorIds\":[\"Out1\"],\"side\":\"RIGHT\"},\"type\":\"ConnectorPlacement.EquallySpacedRectSide\",\"uuid\":\"493db82a-06a2-4a87-b234-4e7c0dd8f89b\"},{\"content\":{\"side\":\"TOP\"},\"type\":\"ConnectorPlacement.EquallySpacedRectSide\",\"uuid\":\"00eff750-16ab-4a5d-887e-7c480e5e0d14\"}]},\"type\":\"ConnectorPlacement.EquallySpacedConnector\",\"uuid\":\"9358f970-c1dc-48f9-b6f8-bcc3c6345ab1\"}],\"packageUris\":[\"http://schema.mathworks.com/mf0/Connector/R2020b\"],\"version\":\"1.0\"}"
  + : PMIOPort  Side=Left
  - : PMIOPort  Port=2  Side=Left
  Udc : Outport
  wires:
  混合三电平子模块1/1(Udc) -> Mux1/1
  Mux1/1 -> Udc/1
  混合三电平子模块5/1(Udc) -> Mux1/5
  混合三电平子模块4/1(Udc) -> Mux1/4
  混合三电平子模块2/1(Udc) -> Mux1/2
  混合三电平子模块3/1(Udc) -> Mux1/3
  Demux1/5 -> 混合三电平子模块5/1(DRV)
  Demux1/4 -> 混合三电平子模块4/1(DRV)
  Demux1/2 -> 混合三电平子模块2/1(DRV)
  Demux1/3 -> 混合三电平子模块3/1(DRV)
  Demux1/1 -> 混合三电平子模块1/1(DRV)
  DRV/1 -> Demux1/1
  connections:
  混合三电平子模块5/LConn1 -- 混合三电平子模块4/LConn2
  混合三电平子模块4/LConn1 -- 混合三电平子模块3/LConn2
  混合三电平子模块3/LConn1 -- 混合三电平子模块2/LConn2
  混合三电平子模块2/LConn1 -- 混合三电平子模块1/LConn2
  +/RConn1 -- 混合三电平子模块1/LConn1
  混合三电平子模块5/LConn2 -- -/RConn1

== system MMC_21_Level_Rectifier/三电平级联混合MMC/Subsystem3/Subsystem ==
  DRV : Inport
  Demux1 : Demux  Outputs=5
  Mux1 : Mux  Inputs=5
  混合三电平子模块1 : Subsystem
      settings: PortSchema="{\"entries\":[{\"content\":{\"sides\":[{\"content\":{\"connectorIds\":[\"LConn1\",\"In1\",\"LConn2\"]},\"type\":\"ConnectorPlacement.EquallySpacedRectSide\",\"uuid\":\"9e595762-cb5d-4bdb-b148-c61b2a1e03b2\"},{\"content\":{\"connectorIds\":[\"Out1\"],\"side\":\"RIGHT\"},\"type\":\"ConnectorPlacement.EquallySpacedRectSide\",\"uuid\":\"493db82a-06a2-4a87-b234-4e7c0dd8f89b\"},{\"content\":{\"side\":\"TOP\"},\"type\":\"ConnectorPlacement.EquallySpacedRectSide\",\"uuid\":\"00eff750-16ab-4a5d-887e-7c480e5e0d14\"}]},\"type\":\"ConnectorPlacement.EquallySpacedConnector\",\"uuid\":\"9358f970-c1dc-48f9-b6f8-bcc3c6345ab1\"}],\"packageUris\":[\"http://schema.mathworks.com/mf0/Connector/R2020b\"],\"version\":\"1.0\"}"
  混合三电平子模块2 : Subsystem
      settings: PortSchema="{\"entries\":[{\"content\":{\"sides\":[{\"content\":{\"connectorIds\":[\"LConn1\",\"In1\",\"LConn2\"]},\"type\":\"ConnectorPlacement.EquallySpacedRectSide\",\"uuid\":\"9e595762-cb5d-4bdb-b148-c61b2a1e03b2\"},{\"content\":{\"connectorIds\":[\"Out1\"],\"side\":\"RIGHT\"},\"type\":\"ConnectorPlacement.EquallySpacedRectSide\",\"uuid\":\"493db82a-06a2-4a87-b234-4e7c0dd8f89b\"},{\"content\":{\"side\":\"TOP\"},\"type\":\"ConnectorPlacement.EquallySpacedRectSide\",\"uuid\":\"00eff750-16ab-4a5d-887e-7c480e5e0d14\"}]},\"type\":\"ConnectorPlacement.EquallySpacedConnector\",\"uuid\":\"9358f970-c1dc-48f9-b6f8-bcc3c6345ab1\"}],\"packageUris\":[\"http://schema.mathworks.com/mf0/Connector/R2020b\"],\"version\":\"1.0\"}"
  混合三电平子模块3 : Subsystem
      settings: PortSchema="{\"entries\":[{\"content\":{\"sides\":[{\"content\":{\"connectorIds\":[\"LConn1\",\"In1\",\"LConn2\"]},\"type\":\"ConnectorPlacement.EquallySpacedRectSide\",\"uuid\":\"9e595762-cb5d-4bdb-b148-c61b2a1e03b2\"},{\"content\":{\"connectorIds\":[\"Out1\"],\"side\":\"RIGHT\"},\"type\":\"ConnectorPlacement.EquallySpacedRectSide\",\"uuid\":\"493db82a-06a2-4a87-b234-4e7c0dd8f89b\"},{\"content\":{\"side\":\"TOP\"},\"type\":\"ConnectorPlacement.EquallySpacedRectSide\",\"uuid\":\"00eff750-16ab-4a5d-887e-7c480e5e0d14\"}]},\"type\":\"ConnectorPlacement.EquallySpacedConnector\",\"uuid\":\"9358f970-c1dc-48f9-b6f8-bcc3c6345ab1\"}],\"packageUris\":[\"http://schema.mathworks.com/mf0/Connector/R2020b\"],\"version\":\"1.0\"}"
  混合三电平子模块4 : Subsystem
      settings: PortSchema="{\"entries\":[{\"content\":{\"sides\":[{\"content\":{\"connectorIds\":[\"LConn1\",\"In1\",\"LConn2\"]},\"type\":\"ConnectorPlacement.EquallySpacedRectSide\",\"uuid\":\"9e595762-cb5d-4bdb-b148-c61b2a1e03b2\"},{\"content\":{\"connectorIds\":[\"Out1\"],\"side\":\"RIGHT\"},\"type\":\"ConnectorPlacement.EquallySpacedRectSide\",\"uuid\":\"493db82a-06a2-4a87-b234-4e7c0dd8f89b\"},{\"content\":{\"side\":\"TOP\"},\"type\":\"ConnectorPlacement.EquallySpacedRectSide\",\"uuid\":\"00eff750-16ab-4a5d-887e-7c480e5e0d14\"}]},\"type\":\"ConnectorPlacement.EquallySpacedConnector\",\"uuid\":\"9358f970-c1dc-48f9-b6f8-bcc3c6345ab1\"}],\"packageUris\":[\"http://schema.mathworks.com/mf0/Connector/R2020b\"],\"version\":\"1.0\"}"
  混合三电平子模块5 : Subsystem
      settings: PortSchema="{\"entries\":[{\"content\":{\"sides\":[{\"content\":{\"connectorIds\":[\"LConn1\",\"In1\",\"LConn2\"]},\"type\":\"ConnectorPlacement.EquallySpacedRectSide\",\"uuid\":\"9e595762-cb5d-4bdb-b148-c61b2a1e03b2\"},{\"content\":{\"connectorIds\":[\"Out1\"],\"side\":\"RIGHT\"},\"type\":\"ConnectorPlacement.EquallySpacedRectSide\",\"uuid\":\"493db82a-06a2-4a87-b234-4e7c0dd8f89b\"},{\"content\":{\"side\":\"TOP\"},\"type\":\"ConnectorPlacement.EquallySpacedRectSide\",\"uuid\":\"00eff750-16ab-4a5d-887e-7c480e5e0d14\"}]},\"type\":\"ConnectorPlacement.EquallySpacedConnector\",\"uuid\":\"9358f970-c1dc-48f9-b6f8-bcc3c6345ab1\"}],\"packageUris\":[\"http://schema.mathworks.com/mf0/Connector/R2020b\"],\"version\":\"1.0\"}"
  + : PMIOPort  Side=Left
  - : PMIOPort  Port=2  Side=Left
  Udc : Outport
  wires:
  DRV/1 -> Demux1/1
  Demux1/1 -> 混合三电平子模块1/1(DRV)
  Demux1/3 -> 混合三电平子模块3/1(DRV)
  Demux1/2 -> 混合三电平子模块2/1(DRV)
  Demux1/4 -> 混合三电平子模块4/1(DRV)
  Demux1/5 -> 混合三电平子模块5/1(DRV)
  混合三电平子模块3/1(Udc) -> Mux1/3
  混合三电平子模块2/1(Udc) -> Mux1/2
  混合三电平子模块4/1(Udc) -> Mux1/4
  混合三电平子模块5/1(Udc) -> Mux1/5
  Mux1/1 -> Udc/1
  混合三电平子模块1/1(Udc) -> Mux1/1
  connections:
  混合三电平子模块5/LConn2 -- -/RConn1
  +/RConn1 -- 混合三电平子模块1/LConn1
  混合三电平子模块2/LConn1 -- 混合三电平子模块1/LConn2
  混合三电平子模块3/LConn1 -- 混合三电平子模块2/LConn2
  混合三电平子模块4/LConn1 -- 混合三电平子模块3/LConn2
  混合三电平子模块5/LConn1 -- 混合三电平子模块4/LConn2

== system MMC_21_Level_Rectifier/三电平级联混合MMC/Subsystem3/Subsystem1 ==
  DRV : Inport
  Demux1 : Demux  Outputs=5
  Mux1 : Mux  Inputs=5
  混合三电平子模块1 : Subsystem
      settings: PortSchema="{\"entries\":[{\"content\":{\"sides\":[{\"content\":{\"connectorIds\":[\"LConn1\",\"In1\",\"LConn2\"]},\"type\":\"ConnectorPlacement.EquallySpacedRectSide\",\"uuid\":\"9e595762-cb5d-4bdb-b148-c61b2a1e03b2\"},{\"content\":{\"connectorIds\":[\"Out1\"],\"side\":\"RIGHT\"},\"type\":\"ConnectorPlacement.EquallySpacedRectSide\",\"uuid\":\"493db82a-06a2-4a87-b234-4e7c0dd8f89b\"},{\"content\":{\"side\":\"TOP\"},\"type\":\"ConnectorPlacement.EquallySpacedRectSide\",\"uuid\":\"00eff750-16ab-4a5d-887e-7c480e5e0d14\"}]},\"type\":\"ConnectorPlacement.EquallySpacedConnector\",\"uuid\":\"9358f970-c1dc-48f9-b6f8-bcc3c6345ab1\"}],\"packageUris\":[\"http://schema.mathworks.com/mf0/Connector/R2020b\"],\"version\":\"1.0\"}"
  混合三电平子模块2 : Subsystem
      settings: PortSchema="{\"entries\":[{\"content\":{\"sides\":[{\"content\":{\"connectorIds\":[\"LConn1\",\"In1\",\"LConn2\"]},\"type\":\"ConnectorPlacement.EquallySpacedRectSide\",\"uuid\":\"9e595762-cb5d-4bdb-b148-c61b2a1e03b2\"},{\"content\":{\"connectorIds\":[\"Out1\"],\"side\":\"RIGHT\"},\"type\":\"ConnectorPlacement.EquallySpacedRectSide\",\"uuid\":\"493db82a-06a2-4a87-b234-4e7c0dd8f89b\"},{\"content\":{\"side\":\"TOP\"},\"type\":\"ConnectorPlacement.EquallySpacedRectSide\",\"uuid\":\"00eff750-16ab-4a5d-887e-7c480e5e0d14\"}]},\"type\":\"ConnectorPlacement.EquallySpacedConnector\",\"uuid\":\"9358f970-c1dc-48f9-b6f8-bcc3c6345ab1\"}],\"packageUris\":[\"http://schema.mathworks.com/mf0/Connector/R2020b\"],\"version\":\"1.0\"}"
  混合三电平子模块3 : Subsystem
      settings: PortSchema="{\"entries\":[{\"content\":{\"sides\":[{\"content\":{\"connectorIds\":[\"LConn1\",\"In1\",\"LConn2\"]},\"type\":\"ConnectorPlacement.EquallySpacedRectSide\",\"uuid\":\"9e595762-cb5d-4bdb-b148-c61b2a1e03b2\"},{\"content\":{\"connectorIds\":[\"Out1\"],\"side\":\"RIGHT\"},\"type\":\"ConnectorPlacement.EquallySpacedRectSide\",\"uuid\":\"493db82a-06a2-4a87-b234-4e7c0dd8f89b\"},{\"content\":{\"side\":\"TOP\"},\"type\":\"ConnectorPlacement.EquallySpacedRectSide\",\"uuid\":\"00eff750-16ab-4a5d-887e-7c480e5e0d14\"}]},\"type\":\"ConnectorPlacement.EquallySpacedConnector\",\"uuid\":\"9358f970-c1dc-48f9-b6f8-bcc3c6345ab1\"}],\"packageUris\":[\"http://schema.mathworks.com/mf0/Connector/R2020b\"],\"version\":\"1.0\"}"
  混合三电平子模块4 : Subsystem
      settings: PortSchema="{\"entries\":[{\"content\":{\"sides\":[{\"content\":{\"connectorIds\":[\"LConn1\",\"In1\",\"LConn2\"]},\"type\":\"ConnectorPlacement.EquallySpacedRectSide\",\"uuid\":\"9e595762-cb5d-4bdb-b148-c61b2a1e03b2\"},{\"content\":{\"connectorIds\":[\"Out1\"],\"side\":\"RIGHT\"},\"type\":\"ConnectorPlacement.EquallySpacedRectSide\",\"uuid\":\"493db82a-06a2-4a87-b234-4e7c0dd8f89b\"},{\"content\":{\"side\":\"TOP\"},\"type\":\"ConnectorPlacement.EquallySpacedRectSide\",\"uuid\":\"00eff750-16ab-4a5d-887e-7c480e5e0d14\"}]},\"type\":\"ConnectorPlacement.EquallySpacedConnector\",\"uuid\":\"9358f970-c1dc-48f9-b6f8-bcc3c6345ab1\"}],\"packageUris\":[\"http://schema.mathworks.com/mf0/Connector/R2020b\"],\"version\":\"1.0\"}"
  混合三电平子模块5 : Subsystem
      settings: PortSchema="{\"entries\":[{\"content\":{\"sides\":[{\"content\":{\"connectorIds\":[\"LConn1\",\"In1\",\"LConn2\"]},\"type\":\"ConnectorPlacement.EquallySpacedRectSide\",\"uuid\":\"9e595762-cb5d-4bdb-b148-c61b2a1e03b2\"},{\"content\":{\"connectorIds\":[\"Out1\"],\"side\":\"RIGHT\"},\"type\":\"ConnectorPlacement.EquallySpacedRectSide\",\"uuid\":\"493db82a-06a2-4a87-b234-4e7c0dd8f89b\"},{\"content\":{\"side\":\"TOP\"},\"type\":\"ConnectorPlacement.EquallySpacedRectSide\",\"uuid\":\"00eff750-16ab-4a5d-887e-7c480e5e0d14\"}]},\"type\":\"ConnectorPlacement.EquallySpacedConnector\",\"uuid\":\"9358f970-c1dc-48f9-b6f8-bcc3c6345ab1\"}],\"packageUris\":[\"http://schema.mathworks.com/mf0/Connector/R2020b\"],\"version\":\"1.0\"}"
  + : PMIOPort  Side=Left
  - : PMIOPort  Port=2  Side=Left
  Udc : Outport
  wires:
  混合三电平子模块1/1(Udc) -> Mux1/1
  Mux1/1 -> Udc/1
  混合三电平子模块5/1(Udc) -> Mux1/5
  混合三电平子模块4/1(Udc) -> Mux1/4
  混合三电平子模块2/1(Udc) -> Mux1/2
  混合三电平子模块3/1(Udc) -> Mux1/3
  Demux1/5 -> 混合三电平子模块5/1(DRV)
  Demux1/4 -> 混合三电平子模块4/1(DRV)
  Demux1/2 -> 混合三电平子模块2/1(DRV)
  Demux1/3 -> 混合三电平子模块3/1(DRV)
  Demux1/1 -> 混合三电平子模块1/1(DRV)
  DRV/1 -> Demux1/1
  connections:
  混合三电平子模块5/LConn1 -- 混合三电平子模块4/LConn2
  混合三电平子模块4/LConn1 -- 混合三电平子模块3/LConn2
  混合三电平子模块3/LConn1 -- 混合三电平子模块2/LConn2
  混合三电平子模块2/LConn1 -- 混合三电平子模块1/LConn2
  +/RConn1 -- 混合三电平子模块1/LConn1
  混合三电平子模块5/LConn2 -- -/RConn1

== system MMC_21_Level_Rectifier/三电平级联混合MMC/Subsystem1/Subsystem/混合三电平子模块1 ==
  DRV : Inport
  C0 : spsSeriesRLCBranchLib/Series RLC Branch  LConnTagsString=__new0  RConnTagsString=__new0  BranchType=C  Resistance=0.1  Inductance=0  SetiL0=off  InitialCurrent=0  Capacitance=2e-3  Setx0=on  InitialVoltage=2200  Measurements=None
  C1 : spsSeriesRLCBranchLib/Series RLC Branch  LConnTagsString=__new0  RConnTagsString=__new0  BranchType=C  Resistance=0.1  Inductance=0  SetiL0=off  InitialCurrent=0  Capacitance=2e-3  Setx0=on  InitialVoltage=2200  Measurements=None
  Demux3 : Demux  Outputs=2
  Mux : Mux  Inputs=2
  Universal Bridge1 : spsUniversalBridgeLib/Universal Bridge  Arms=1  SnubberResistance=1e6  SnubberCapacitance=inf  Device=IGBT / Diodes  Ron=1e-3  Lon=0  ForwardVoltages="[  1  1  ]"  ForwardVoltage=0  GTOparameters=[ 10e-6 , 20e-6 ]  IGBTparameters=[ 1e-6 , 2e-6 ]  Measurements=None  Measurements_2=None  converterType=Rectifier
  Universal Bridge2 : spsUniversalBridgeLib/Universal Bridge  Arms=1  SnubberResistance=1e6  SnubberCapacitance=inf  Device=IGBT / Diodes  Ron=1e-3  Lon=0  ForwardVoltages="[  1  1  ]"  ForwardVoltage=0  GTOparameters=[ 10e-6 , 20e-6 ]  IGBTparameters=[ 1e-6 , 2e-6 ]  Measurements=None  Measurements_2=None  converterType=Rectifier
  Vm1 : spsVoltageMeasurementLib/Voltage Measurement  PhasorSimulation=off  OutputType=Complex  PSBequivalent=0
  Vm3 : spsVoltageMeasurementLib/Voltage Measurement  PhasorSimulation=off  OutputType=Complex  PSBequivalent=0
  A : PMIOPort  Side=Left
  B : PMIOPort  Port=2  Side=Left
  Udc : Outport
  wires:
  Mux/1 -> Udc/1
  DRV/1 -> Demux3/1
  Demux3/2 -> Universal Bridge2/1
  Vm1/1 -> Mux/1
  Vm3/1 -> Mux/2
  Demux3/1 -> Universal Bridge1/1
  connections:
  Vm1/LConn2 -- C0/RConn1 -- Universal Bridge1/RConn2 -- Universal Bridge2/LConn1
  Universal Bridge1/LConn1 -- A/RConn1
  Vm3/LConn1 -- C1/LConn1 -- Universal Bridge2/RConn1
  Vm1/LConn1 -- Universal Bridge1/RConn1 -- C0/LConn1
  Universal Bridge2/RConn2 -- C1/RConn1 -- B/RConn1 -- Vm3/LConn2

== system MMC_21_Level_Rectifier/三电平级联混合MMC/Subsystem1/Subsystem/混合三电平子模块2 ==
  DRV : Inport
  C0 : spsSeriesRLCBranchLib/Series RLC Branch  LConnTagsString=__new0  RConnTagsString=__new0  BranchType=C  Resistance=0.1  Inductance=0  SetiL0=off  InitialCurrent=0  Capacitance=2e-3  Setx0=on  InitialVoltage=2200  Measurements=None
  C1 : spsSeriesRLCBranchLib/Series RLC Branch  LConnTagsString=__new0  RConnTagsString=__new0  BranchType=C  Resistance=0.1  Inductance=0  SetiL0=off  InitialCurrent=0  Capacitance=2e-3  Setx0=on  InitialVoltage=2200  Measurements=None
  Demux3 : Demux  Outputs=2
  Mux : Mux  Inputs=2
  Universal Bridge1 : spsUniversalBridgeLib/Universal Bridge  Arms=1  SnubberResistance=1e6  SnubberCapacitance=inf  Device=IGBT / Diodes  Ron=1e-3  Lon=0  ForwardVoltages="[  1  1  ]"  ForwardVoltage=0  GTOparameters=[ 10e-6 , 20e-6 ]  IGBTparameters=[ 1e-6 , 2e-6 ]  Measurements=None  Measurements_2=None  converterType=Rectifier
  Universal Bridge2 : spsUniversalBridgeLib/Universal Bridge  Arms=1  SnubberResistance=1e6  SnubberCapacitance=inf  Device=IGBT / Diodes  Ron=1e-3  Lon=0  ForwardVoltages="[  1  1  ]"  ForwardVoltage=0  GTOparameters=[ 10e-6 , 20e-6 ]  IGBTparameters=[ 1e-6 , 2e-6 ]  Measurements=None  Measurements_2=None  converterType=Rectifier
  Vm1 : spsVoltageMeasurementLib/Voltage Measurement  PhasorSimulation=off  OutputType=Complex  PSBequivalent=0
  Vm3 : spsVoltageMeasurementLib/Voltage Measurement  PhasorSimulation=off  OutputType=Complex  PSBequivalent=0
  A : PMIOPort  Side=Left
  B : PMIOPort  Port=2  Side=Left
  Udc : Outport
  wires:
  Demux3/1 -> Universal Bridge1/1
  Vm3/1 -> Mux/2
  Vm1/1 -> Mux/1
  Demux3/2 -> Universal Bridge2/1
  DRV/1 -> Demux3/1
  Mux/1 -> Udc/1
  connections:
  Vm3/LConn2 -- B/RConn1 -- C1/RConn1 -- Universal Bridge2/RConn2
  C0/LConn1 -- Universal Bridge1/RConn1 -- Vm1/LConn1
  Universal Bridge2/RConn1 -- C1/LConn1 -- Vm3/LConn1
  Universal Bridge1/LConn1 -- A/RConn1
  Universal Bridge2/LConn1 -- Universal Bridge1/RConn2 -- C0/RConn1 -- Vm1/LConn2

== system MMC_21_Level_Rectifier/三电平级联混合MMC/Subsystem1/Subsystem/混合三电平子模块3 ==
  DRV : Inport
  C0 : spsSeriesRLCBranchLib/Series RLC Branch  LConnTagsString=__new0  RConnTagsString=__new0  BranchType=C  Resistance=0.1  Inductance=0  SetiL0=off  InitialCurrent=0  Capacitance=2e-3  Setx0=on  InitialVoltage=2200  Measurements=None
  C1 : spsSeriesRLCBranchLib/Series RLC Branch  LConnTagsString=__new0  RConnTagsString=__new0  BranchType=C  Resistance=0.1  Inductance=0  SetiL0=off  InitialCurrent=0  Capacitance=2e-3  Setx0=on  InitialVoltage=2200  Measurements=None
  Demux3 : Demux  Outputs=2
  Mux : Mux  Inputs=2
  Universal Bridge1 : spsUniversalBridgeLib/Universal Bridge  Arms=1  SnubberResistance=1e6  SnubberCapacitance=inf  Device=IGBT / Diodes  Ron=1e-3  Lon=0  ForwardVoltages="[  1  1  ]"  ForwardVoltage=0  GTOparameters=[ 10e-6 , 20e-6 ]  IGBTparameters=[ 1e-6 , 2e-6 ]  Measurements=None  Measurements_2=None  converterType=Rectifier
  Universal Bridge2 : spsUniversalBridgeLib/Universal Bridge  Arms=1  SnubberResistance=1e6  SnubberCapacitance=inf  Device=IGBT / Diodes  Ron=1e-3  Lon=0  ForwardVoltages="[  1  1  ]"  ForwardVoltage=0  GTOparameters=[ 10e-6 , 20e-6 ]  IGBTparameters=[ 1e-6 , 2e-6 ]  Measurements=None  Measurements_2=None  converterType=Rectifier
  Vm1 : spsVoltageMeasurementLib/Voltage Measurement  PhasorSimulation=off  OutputType=Complex  PSBequivalent=0
  Vm3 : spsVoltageMeasurementLib/Voltage Measurement  PhasorSimulation=off  OutputType=Complex  PSBequivalent=0
  A : PMIOPort  Side=Left
  B : PMIOPort  Port=2  Side=Left
  Udc : Outport
  wires:
  Mux/1 -> Udc/1
  DRV/1 -> Demux3/1
  Demux3/2 -> Universal Bridge2/1
  Vm1/1 -> Mux/1
  Vm3/1 -> Mux/2
  Demux3/1 -> Universal Bridge1/1
  connections:
  Vm1/LConn2 -- C0/RConn1 -- Universal Bridge1/RConn2 -- Universal Bridge2/LConn1
  Universal Bridge1/LConn1 -- A/RConn1
  Vm3/LConn1 -- C1/LConn1 -- Universal Bridge2/RConn1
  Vm1/LConn1 -- Universal Bridge1/RConn1 -- C0/LConn1
  Universal Bridge2/RConn2 -- C1/RConn1 -- B/RConn1 -- Vm3/LConn2

== system MMC_21_Level_Rectifier/三电平级联混合MMC/Subsystem1/Subsystem/混合三电平子模块4 ==
  DRV : Inport
  C0 : spsSeriesRLCBranchLib/Series RLC Branch  LConnTagsString=__new0  RConnTagsString=__new0  BranchType=C  Resistance=0.1  Inductance=0  SetiL0=off  InitialCurrent=0  Capacitance=2e-3  Setx0=on  InitialVoltage=2200  Measurements=None
  C1 : spsSeriesRLCBranchLib/Series RLC Branch  LConnTagsString=__new0  RConnTagsString=__new0  BranchType=C  Resistance=0.1  Inductance=0  SetiL0=off  InitialCurrent=0  Capacitance=2e-3  Setx0=on  InitialVoltage=2200  Measurements=None
  Demux3 : Demux  Outputs=2
  Mux : Mux  Inputs=2
  Universal Bridge1 : spsUniversalBridgeLib/Universal Bridge  Arms=1  SnubberResistance=1e6  SnubberCapacitance=inf  Device=IGBT / Diodes  Ron=1e-3  Lon=0  ForwardVoltages="[  1  1  ]"  ForwardVoltage=0  GTOparameters=[ 10e-6 , 20e-6 ]  IGBTparameters=[ 1e-6 , 2e-6 ]  Measurements=None  Measurements_2=None  converterType=Rectifier
  Universal Bridge2 : spsUniversalBridgeLib/Universal Bridge  Arms=1  SnubberResistance=1e6  SnubberCapacitance=inf  Device=IGBT / Diodes  Ron=1e-3  Lon=0  ForwardVoltages="[  1  1  ]"  ForwardVoltage=0  GTOparameters=[ 10e-6 , 20e-6 ]  IGBTparameters=[ 1e-6 , 2e-6 ]  Measurements=None  Measurements_2=None  converterType=Rectifier
  Vm1 : spsVoltageMeasurementLib/Voltage Measurement  PhasorSimulation=off  OutputType=Complex  PSBequivalent=0
  Vm3 : spsVoltageMeasurementLib/Voltage Measurement  PhasorSimulation=off  OutputType=Complex  PSBequivalent=0
  A : PMIOPort  Side=Left
  B : PMIOPort  Port=2  Side=Left
  Udc : Outport
  wires:
  Demux3/1 -> Universal Bridge1/1
  Vm3/1 -> Mux/2
  Vm1/1 -> Mux/1
  Demux3/2 -> Universal Bridge2/1
  DRV/1 -> Demux3/1
  Mux/1 -> Udc/1
  connections:
  Vm3/LConn2 -- B/RConn1 -- C1/RConn1 -- Universal Bridge2/RConn2
  C0/LConn1 -- Universal Bridge1/RConn1 -- Vm1/LConn1
  Universal Bridge2/RConn1 -- C1/LConn1 -- Vm3/LConn1
  Universal Bridge1/LConn1 -- A/RConn1
  Universal Bridge2/LConn1 -- Universal Bridge1/RConn2 -- C0/RConn1 -- Vm1/LConn2
